simulink model "HRES_ORC_PEM"  (R2025b)
settings: Solver=ode23t  StartTime=0.0  StopTime=35000  MaxStep=1728  RelTol=1e-3
model workspace (MAT data in the model file):
  CND_L = 10
  CND_T0 = 333.15
  CND_d = 0.012
  CND_n = 20
  CND_p0 = 150000
  GAS_Tmax = 430
  GAS_dT = 20
  GAS_kb = 0.04
  GAS_ki = 0.002
  GAS_kp = 0.05
  GAS_min = 0.02
  GAS_total = 5
  GAS_u0 = 0.05
  HRS_L = 10
  HRS_LG = 1
  HRS_d = 0.012
  HRS_n = 6
  HRS_nG = 25
  HRS_p0 = 0.3
  HRS_x0 = 0.2
  NOZ_kb = 0.025
  NOZ_ki = 0.0005
  NOZ_kp = 0.02
  NOZ_min = 0.01
  NOZ_u0 = 0.1
  ORC_T3set = 400
  ORC_Taux = -2
  ORC_Taux0 = 0
  ORC_kb = 0.4
  ORC_ki = 2e-07
  ORC_kp = 5e-07
  ORC_mdot0 = 0.2
  ORC_mmax = 1
  ORC_mmin = 0.01
  ORC_pset_MPa = 1
  RCV_V = 0.2
  RCV_frac0 = 0.5
  RCV_p0 = 0.15
  RCV_tau = 0.1
  TRB_Tref = 400
  TRB_mdot = 0.6
  TRB_pr = 6
values from neighbouring files (symbols this model uses):
  R_h2 = 4.12    [run_simulation.m]
libraries: fl_lib x62, nesl_utility x56, SimscapeFluids_lib x9, slpidlib x4, ee_lib x2
(part 3 of 5)

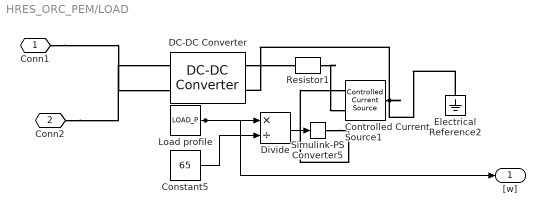
== system HRES_ORC_PEM/LOAD ==
  Constant5 : Constant  Value=65
  Controlled Current Source1 : fl_lib/Electrical/Electrical Sources/Controlled Current Source
  DC-DC Converter : ee_lib/Semiconductors & Converters/Converters/DC-DC Converter  Vref_option=ee.enum.converters.voltageref.internal  v_ref=65 V  P_rated=10 kW  droop_enabled=true  droop_param=ee.enum.converters.droop.value  droop=0.1 V/A  droop_percent=2  Vref_droop=10 V  reversible=ee.enum.converters.directionality.unidirectional  G_diode=1e-8 1/Ohm  P_fixed=1 W  losses_option=ee.enum.converters.lossesOption.proportionalToSquaredCurrent  eff_rated=80  tableOption=ee.enum.converters.lossTableOptionThermal.currentTemp  i_eff_vec=[-2, -1, 1, 2] A  v_eff_vec=[15, 30, 45] V  eff_vec=[66, 76, 80, 74]  eff_2D_table=[66, 66, 66; 76, 76, 76; 80, 80, 80; 74, 74, 74]  model_dynamics=ee.enum.converters.dynamics.no  tau=0.02 s  v_ini=10 V  v1_min=1 V  R1=1000 Ohm  R2=1000 Ohm  fault_condition=ee.enum.faults.faultInputCondition.greaterThan  fault_threshold=0.5  T_eff_vec=[280, 300, 320] K  eff_3D_table=repmat([66; 76; 80; 74], 1, 3, 3)  thermal_mass=100 J/K  initial_temperature=298.15 K
      settings: InternalSimscapePortConfiguration="{\"Bottom\":[],\"Left\":[{\"id\":\"p1\",\"label\":\"1+\",\"type\":\"foundation.electrical.electrical\"},{\"id\":\"n1\",\"label\":\"1-\",\"type\":\"foundation.electrical.electrical\"}],\"Right\":[{\"id\":\"p2\",\"label\":\"2+\",\"type\":\"foundation.electrical.electrical\"},{\"id\":\"n2\",\"label\":\"2-\",\"type\":\"foundation.electrical.electrical\"}],\"Top\":[]}"
  Divide : Product  Inputs=*/
  Electrical Reference2 : fl_lib/Electrical/Electrical Elements/Electrical Reference
  Load profile : FromWorkspace  VariableName=LOAD_P  OutputAfterFinalValue=Holding final value
  Resistor1 : fl_lib/Electrical/Electrical Elements/Resistor  R=0.1 Ohm  i_specify=off  i_priority=None  i=0 A  i_nominal_specify=off  i_nominal_value=1  i_nominal_unit=A  v_specify=off  v_priority=None  v=0 V  v_nominal_specify=off  v_nominal_value=1  v_nominal_unit=V
  Simulink-PS Converter5 : nesl_utility/Simulink-PS Converter  PhysicalDomain=network_engine_domain  SubClassName=ps_input  LeftPortType=input  RightPortType=output  PseudoPeriodic=off  Frequencies=[]  NoiseDistribution=none  NoiseParameters=[]  Unit=1  AffineConversion=off  FilteringAndDerivatives=provide  SimscapeFilterOrder=1  InputFilterTimeConstant=0.001  UdotUserProvided=0
  Conn1 : PMIOPort  Side=Left
  Conn2 : PMIOPort  Port=2  Side=Left
  "[w]" : Outport
  wires:
  Divide/1 -> Simulink-PS Converter5/1
  Constant5/1 -> Divide/2
  Load profile/1 -> "[w]"/1, Divide/1
  connections:
  Conn1/RConn1 -- DC-DC Converter/LConn2
  Resistor1/RConn1 -- Controlled Current Source1/RConn2
  DC-DC Converter/RConn1 -- Resistor1/LConn1
  Simulink-PS Converter5/RConn1 -- Controlled Current Source1/RConn1
  Controlled Current Source1/LConn1 -- Electrical Reference2/LConn1 -- DC-DC Converter/RConn2
  Conn2/RConn1 -- DC-DC Converter/LConn1
